simulink model "gm_PMLSM_FOC_FixedPoint_vnl"  (R2026b)
settings: Solver=FixedStepDiscrete  StopTime=0.0063  FixedStep=2e-08
undefined symbols (not defined in the file): FOC_Fixed_Config, Lookup, Ts_ACR
libraries: hdlmdlgenlib x38, simulink x16, mcbeeMathTransformLib x2
(part 2 of 6)

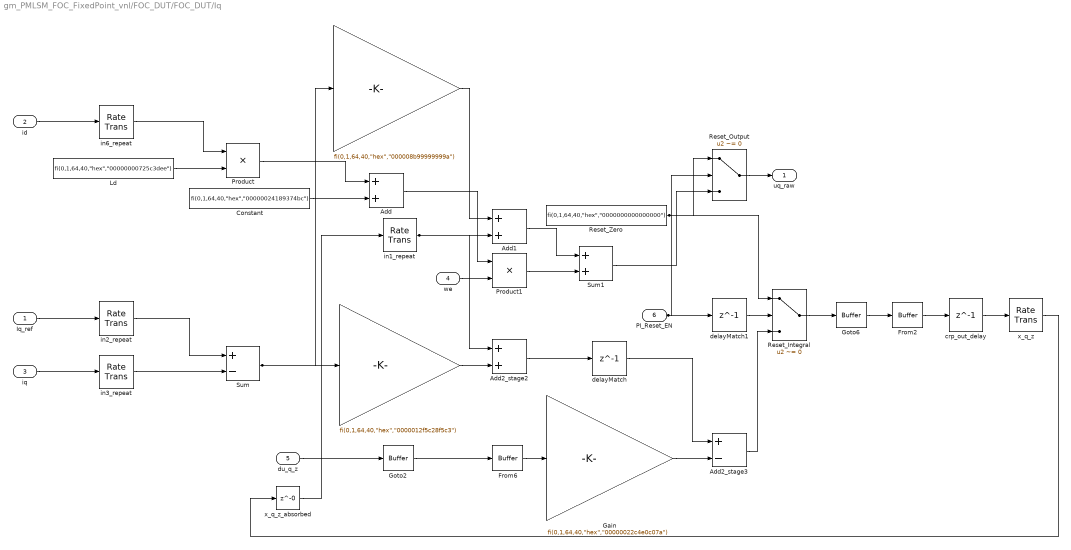
== system gm_PMLSM_FOC_FixedPoint_vnl/FOC_DUT/FOC_DUT/Iq ==
  Iq_ref : Inport  OutDataTypeStr=fixdt(1, 32, 24)  PortDimensions=1  SampleTime=0.0001
  id : Inport  Port=2  OutDataTypeStr=fixdt(1, 64, 40)  PortDimensions=1  SampleTime=0.0001
  iq : Inport  Port=3  OutDataTypeStr=fixdt(1, 64, 40)  PortDimensions=1  SampleTime=0.0001
  we : Inport  Port=4  OutDataTypeStr=fixdt(1, 40, 24)  PortDimensions=1  SampleTime=2e-08
  du_q_z : Inport  Port=5  OutDataTypeStr=fixdt(1, 64, 40)  PortDimensions=1  SampleTime=2e-08
  PI_Reset_EN : Inport  Port=6  OutDataTypeStr=boolean  PortDimensions=1  SampleTime=2e-08
  " " : Gain  Gain="fi(0,1,64,40,\"hex\",\"0000012f5c28f5c3\")"  ParamDataTypeStr=fixdt(1, 64, 40)  OutDataTypeStr=fixdt(1, 64, 40)  RndMeth=Convergent  SaturateOnIntegerOverflow=on  SampleTime=2e-08
  "  " : Gain  Gain="fi(0,1,64,40,\"hex\",\"000008b99999999a\")"  ParamDataTypeStr=fixdt(1, 64, 40)  OutDataTypeStr=fixdt(1, 64, 40)  RndMeth=Convergent  SaturateOnIntegerOverflow=on  SampleTime=2e-08
  Add : Sum  OutDataTypeStr=fixdt(1, 64, 40)  AccumDataTypeStr=fixdt(1, 64, 40)  RndMeth=Convergent  SaturateOnIntegerOverflow=on  SampleTime=2e-08
  Add1 : Sum  OutDataTypeStr=fixdt(1, 64, 40)  AccumDataTypeStr=fixdt(1, 64, 40)  RndMeth=Convergent  SaturateOnIntegerOverflow=on  SampleTime=2e-08
  Add2_stage2 : Sum  OutDataTypeStr=fixdt(1, 64, 40)  AccumDataTypeStr=fixdt(1, 64, 40)  RndMeth=Convergent  SaturateOnIntegerOverflow=on  SampleTime=2e-08
  Add2_stage3 : Sum  Inputs=+-  OutDataTypeStr=fixdt(1, 64, 40)  AccumDataTypeStr=fixdt(1, 64, 40)  RndMeth=Convergent  SaturateOnIntegerOverflow=on  SampleTime=2e-08
  Constant : Constant  Value="fi(0,1,64,40,\"hex\",\"00000024189374bc\")"  OutDataTypeStr=fixdt(1, 64, 40)  SampleTime=2e-08
  From2 : hdlmdlgenlib/Buffer
  From6 : hdlmdlgenlib/Buffer
  Gain : Gain  Gain="fi(0,1,64,40,\"hex\",\"00000022c4e0c07a\")"  ParamDataTypeStr=fixdt(1, 64, 40)  OutDataTypeStr=fixdt(1, 64, 40)  RndMeth=Convergent  SaturateOnIntegerOverflow=on  SampleTime=2e-08
  Goto2 : hdlmdlgenlib/Buffer
  Goto6 : hdlmdlgenlib/Buffer
  Ld : Constant  Value="fi(0,1,64,40,\"hex\",\"00000000725c3dee\")"  OutDataTypeStr=fixdt(1, 64, 40)  SampleTime=2e-08
  Product : Product  Inputs=**  OutDataTypeStr=fixdt(1, 64, 40)  RndMeth=Convergent  SaturateOnIntegerOverflow=on  SampleTime=2e-08
  Product1 : Product  Inputs=**  OutDataTypeStr=fixdt(1, 64, 40)  RndMeth=Convergent  SaturateOnIntegerOverflow=on  SampleTime=2e-08
  Reset_Integral : Switch  Criteria=u2 ~= 0  Threshold="fi(0,0,1,0,\"hex\",\"0\")"  OutDataTypeStr=fixdt(1, 64, 40)  RndMeth=Convergent  SampleTime=2e-08  InputSameDT=off
  Reset_Output : Switch  Criteria=u2 ~= 0  Threshold="fi(0,0,1,0,\"hex\",\"0\")"  OutDataTypeStr=fixdt(1, 64, 40)  RndMeth=Convergent  SampleTime=2e-08  InputSameDT=off
  Reset_Zero : Constant  Value="fi(0,1,64,40,\"hex\",\"0000000000000000\")"  OutDataTypeStr=fixdt(1, 64, 40)  SampleTime=2e-08
  Sum : Sum  Inputs=+-  OutDataTypeStr=fixdt(1, 64, 40)  AccumDataTypeStr=fixdt(1, 64, 40)  RndMeth=Convergent  SaturateOnIntegerOverflow=on  SampleTime=2e-08
  Sum1 : Sum  OutDataTypeStr=fixdt(1, 64, 40)  AccumDataTypeStr=fixdt(1, 64, 40)  RndMeth=Convergent  SaturateOnIntegerOverflow=on  SampleTime=2e-08
  crp_out_delay : Delay  DelayLength=1  InitialCondition=0  SampleTime=2e-08
  delayMatch : Delay  DelayLength=1  InitialCondition=0  SampleTime=2e-08
  delayMatch1 : Delay  DelayLength=1  InitialCondition=0  SampleTime=2e-08
  in1_repeat : RateTransition  Integrity=off  Deterministic=off  OutPortSampleTimeOpt=Multiple of input port sample time  OutPortSampleTimeMultiple=1/5000
  in2_repeat : RateTransition  Integrity=off  Deterministic=off  OutPortSampleTimeOpt=Multiple of input port sample time  OutPortSampleTimeMultiple=1/5000
  in3_repeat : RateTransition  Integrity=off  Deterministic=off  OutPortSampleTimeOpt=Multiple of input port sample time  OutPortSampleTimeMultiple=1/5000
  in6_repeat : RateTransition  Integrity=off  Deterministic=off  OutPortSampleTimeOpt=Multiple of input port sample time  OutPortSampleTimeMultiple=1/5000
  x_q_z : RateTransition  OutPortSampleTimeOpt=Multiple of input port sample time  OutPortSampleTimeMultiple=5000
  x_q_z_absorbed : Delay  DelayLength=0
  uq_raw : Outport  OutDataTypeStr=fixdt(1, 64, 40)  PortDimensions=1  SampleTime=2e-08
  wires:
  x_q_z/1 -> x_q_z_absorbed/1
  From2/1 -> crp_out_delay/1
  Goto6/1 -> From2/1
  Reset_Integral/1 -> Goto6/1
  Add2_stage3/1 -> Reset_Integral/3
  Gain/1 -> Add2_stage3/2
  delayMatch/1 -> Add2_stage3/1
  PI_Reset_EN/1 -> Reset_Output/2, delayMatch1/1
  Sum1/1 -> Reset_Output/3
  Reset_Zero/1 -> Reset_Output/1, Reset_Integral/1
  From6/1 -> Gain/1
  Add2_stage2/1 -> delayMatch/1
  crp_out_delay/1 -> x_q_z/1
  Product1/1 -> Sum1/2
  Add1/1 -> Sum1/1
  Goto2/1 -> From6/1
  " "/1 -> Add2_stage2/2
  we/1 -> Product1/2
  in1_repeat/1 -> Add1/2, Add2_stage2/1
  Add/1 -> Product1/1
  "  "/1 -> Add1/1
  x_q_z_absorbed/1 -> in1_repeat/1
  du_q_z/1 -> Goto2/1
  Sum/1 -> "  "/1, " "/1
  delayMatch1/1 -> Reset_Integral/2
  Constant/1 -> Add/2
  in3_repeat/1 -> Sum/2
  in2_repeat/1 -> Sum/1
  Product/1 -> Add/1
  iq/1 -> in3_repeat/1
  Iq_ref/1 -> in2_repeat/1
  Reset_Output/1 -> uq_raw/1
  in6_repeat/1 -> Product/1
  id/1 -> in6_repeat/1
  Ld/1 -> Product/2

== system gm_PMLSM_FOC_FixedPoint_vnl/FOC_DUT/FOC_DUT/Park ==
  A : Inport  OutDataTypeStr=fixdt(1,64,40,'DataTypeOverride', 'Off')  PortDimensions=1  SampleTime=0.0001
  B : Inport  Port=2  OutDataTypeStr=fixdt(1,64,40,'DataTypeOverride', 'Off')  PortDimensions=1  SampleTime=0.0001
  C : Inport  Port=3  OutDataTypeStr=fixdt(1,40,32,'DataTypeOverride', 'Off')  PortDimensions=1  SampleTime=0.0001
  Variant : Subsystem
  O1 : Outport  OutDataTypeStr=fixdt(1, 64, 40)  PortDimensions=1  SampleTime=0.0001
  O2 : Outport  Port=2  OutDataTypeStr=fixdt(1, 64, 40)  PortDimensions=1  SampleTime=0.0001
  wires:
  Variant/2(O2) -> O2/1
  C/1 -> Variant/3(C)
  B/1 -> Variant/2(B)
  A/1 -> Variant/1(A)
  Variant/1(O1) -> O1/1

== system gm_PMLSM_FOC_FixedPoint_vnl/FOC_DUT/FOC_DUT/SVPWMG ==
  Valpha : Inport  OutDataTypeStr=fixdt(1, 64, 40)  PortDimensions=1  SampleTime=2e-08
  Vbeta : Inport  Port=2  OutDataTypeStr=fixdt(1, 64, 40)  PortDimensions=1  SampleTime=2e-08
  Vdc_V : Inport  Port=3  OutDataTypeStr=fixdt(0, 32, 24)  PortDimensions=1  SampleTime=2e-08
  Duty Calculate : Subsystem
  Sector Caculate : Subsystem
  T1T2 Calculate : Subsystem
  XYZ Calculate : Subsystem
  duty_u_cmd : Outport  OutDataTypeStr=fixdt(1, 64, 40)  PortDimensions=1  SampleTime=2e-08
  duty_v_cmd : Outport  Port=2  OutDataTypeStr=fixdt(1, 64, 40)  PortDimensions=1  SampleTime=2e-08
  duty_w_cmd : Outport  Port=3  OutDataTypeStr=fixdt(1, 64, 40)  PortDimensions=1  SampleTime=2e-08
  wires:
  Duty Calculate/2(Duty_V) -> duty_v_cmd/1
  Duty Calculate/1(Duty_U) -> duty_u_cmd/1
  T1T2 Calculate/2(T2) -> Duty Calculate/3(T2)
  T1T2 Calculate/1(T1) -> Duty Calculate/2(T1)
  XYZ Calculate/1(X) -> T1T2 Calculate/2(X)
  Vdc_V/1 -> XYZ Calculate/3(Udc)
  Sector Caculate/1("N ") -> T1T2 Calculate/1(N), Duty Calculate/1(N)
  XYZ Calculate/3(Z) -> T1T2 Calculate/4(Z)
  Vbeta/1 -> XYZ Calculate/2(Ubeta), Sector Caculate/2(Ubeta)
  XYZ Calculate/2(Y) -> T1T2 Calculate/3(Y)
  Duty Calculate/3(Duty_W) -> duty_w_cmd/1
  Valpha/1 -> Sector Caculate/1(Ualpha), XYZ Calculate/1(Ualpha)

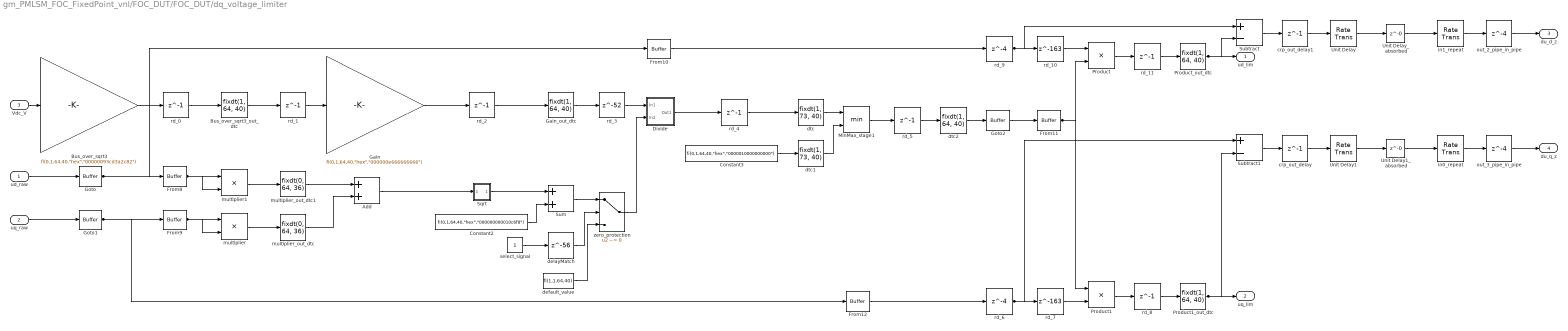
== system gm_PMLSM_FOC_FixedPoint_vnl/FOC_DUT/FOC_DUT/dq_voltage_limiter ==
  ud_raw : Inport  OutDataTypeStr=fixdt(1, 64, 40)  PortDimensions=1  SampleTime=2e-08
  uq_raw : Inport  Port=2  OutDataTypeStr=fixdt(1, 64, 40)  PortDimensions=1  SampleTime=2e-08
  Vdc_V : Inport  Port=3  OutDataTypeStr=fixdt(0, 32, 24)  PortDimensions=1  SampleTime=2e-08
  Add : Sum  OutDataTypeStr=fixdt(0, 64, 36)  AccumDataTypeStr=fixdt(0, 64, 36)  RndMeth=Convergent  SaturateOnIntegerOverflow=on  SampleTime=2e-08
  Bus_over_sqrt3 : Gain  Gain="fi(0,1,64,40,\"hex\",\"00000093cd3a2c82\")"  ParamDataTypeStr=fixdt(1, 64, 40)  OutDataTypeStr=fixdt(1, 96, 64)  SampleTime=2e-08
  Bus_over_sqrt3_out_dtc : DataTypeConversion  OutDataTypeStr=fixdt(1, 64, 40)  RndMeth=Convergent  SampleTime=2e-08
  Constant2 : Constant  Value="fi(0,1,64,40,\"hex\",\"000000000010c6f8\")"  OutDataTypeStr=fixdt(1, 64, 40)  SampleTime=2e-08
  Constant3 : Constant  Value="fi(0,1,64,40,\"hex\",\"0000010000000000\")"  OutDataTypeStr=fixdt(1, 64, 40)  SampleTime=2e-08
  Divide : Subsystem
  From{8..12} (5 alike) : hdlmdlgenlib/Buffer
  Gain : Gain  Gain="fi(0,1,64,40,\"hex\",\"000000e666666666\")"  ParamDataTypeStr=fixdt(1, 64, 40)  OutDataTypeStr=fixdt(1, 128, 80)  SampleTime=2e-08
  Gain_out_dtc : DataTypeConversion  OutDataTypeStr=fixdt(1, 64, 40)  RndMeth=Convergent  SampleTime=2e-08
  Goto : hdlmdlgenlib/Buffer
  Goto1 : hdlmdlgenlib/Buffer
  Goto2 : hdlmdlgenlib/Buffer
  MinMax_stage1 : MinMax  Inputs=2
  Product : Product  Inputs=**  OutDataTypeStr=fixdt(1, 128, 80)  SampleTime=2e-08
  Product1 : Product  Inputs=**  OutDataTypeStr=fixdt(1, 128, 80)  SampleTime=2e-08
  Product1_out_dtc : DataTypeConversion  OutDataTypeStr=fixdt(1, 64, 40)  RndMeth=Convergent  SampleTime=2e-08
  Product_out_dtc : DataTypeConversion  OutDataTypeStr=fixdt(1, 64, 40)  RndMeth=Convergent  SampleTime=2e-08
  Sqrt : Subsystem
  Subtract : Sum  Inputs=+-  OutDataTypeStr=fixdt(1, 64, 40)  AccumDataTypeStr=fixdt(1, 64, 40)  RndMeth=Convergent  SaturateOnIntegerOverflow=on  SampleTime=2e-08
  Subtract1 : Sum  Inputs=+-  OutDataTypeStr=fixdt(1, 64, 40)  AccumDataTypeStr=fixdt(1, 64, 40)  RndMeth=Convergent  SaturateOnIntegerOverflow=on  SampleTime=2e-08
  Sum : Sum  OutDataTypeStr=fixdt(1, 64, 40)  AccumDataTypeStr=fixdt(1, 64, 40)  RndMeth=Convergent  SaturateOnIntegerOverflow=on  SampleTime=2e-08
  Unit Delay : RateTransition  OutPortSampleTimeOpt=Multiple of input port sample time  OutPortSampleTimeMultiple=5000
  Unit Delay1 : RateTransition  OutPortSampleTimeOpt=Multiple of input port sample time  OutPortSampleTimeMultiple=5000
  Unit Delay1_absorbed : Delay  DelayLength=0
  Unit Delay_absorbed : Delay  DelayLength=0
  crp_out_delay : Delay  DelayLength=1  InitialCondition=0  SampleTime=2e-08
  crp_out_delay1 : Delay  DelayLength=1  InitialCondition=0  SampleTime=2e-08
  default_value : Constant  Value=fi(1,1,64,40)  OutDataTypeStr=fixdt(1, 64, 40)  SampleTime=2e-08
  delayMatch : Delay  DelayLength=56  InitialCondition=0  SampleTime=2e-08
  dtc : DataTypeConversion  OutDataTypeStr=fixdt(1, 73, 40)  RndMeth=Convergent  SampleTime=2e-08
  dtc1 : DataTypeConversion  OutDataTypeStr=fixdt(1, 73, 40)  RndMeth=Convergent  SampleTime=2e-08
  dtc2 : DataTypeConversion  OutDataTypeStr=fixdt(1, 64, 40)  RndMeth=Convergent  SampleTime=2e-08
  in0_repeat : RateTransition  Integrity=off  Deterministic=off  OutPortSampleTimeOpt=Multiple of input port sample time  OutPortSampleTimeMultiple=1/5000
  in1_repeat : RateTransition  Integrity=off  Deterministic=off  OutPortSampleTimeOpt=Multiple of input port sample time  OutPortSampleTimeMultiple=1/5000
  multiplier : Product  Inputs=**  OutDataTypeStr=fixdt(1, 128, 80)  SampleTime=2e-08
  multiplier1 : Product  Inputs=**  OutDataTypeStr=fixdt(1, 128, 80)  SampleTime=2e-08
  multiplier_out_dtc : DataTypeConversion  OutDataTypeStr=fixdt(0, 64, 36)  RndMeth=Convergent  SampleTime=2e-08
  multiplier_out_dtc1 : DataTypeConversion  OutDataTypeStr=fixdt(0, 64, 36)  RndMeth=Convergent  SampleTime=2e-08
  out_2_pipe_in_pipe : Delay  DelayLength=4  InitialCondition=0  SampleTime=2e-08
  out_3_pipe_in_pipe : Delay  DelayLength=4  InitialCondition=0  SampleTime=2e-08
  rd_{0..2,4..5,8,11} (7 alike) : Delay  DelayLength=1  InitialCondition=0  SampleTime=2e-08
  rd_10 : Delay  DelayLength=163  InitialCondition=0  SampleTime=2e-08
  rd_3 : Delay  DelayLength=52  InitialCondition=0  SampleTime=2e-08
  rd_6 : Delay  DelayLength=4  InitialCondition=0  SampleTime=2e-08
  rd_7 : Delay  DelayLength=163  InitialCondition=0  SampleTime=2e-08
  rd_9 : Delay  DelayLength=4  InitialCondition=0  SampleTime=2e-08
  select_signal : Constant  OutDataTypeStr=boolean  SampleTime=2e-08
  zero_protection : Switch  Criteria=u2 ~= 0  OutDataTypeStr=fixdt(1, 64, 40)  SampleTime=2e-08  SaturateOnIntegerOverflow=off  InputSameDT=off
  ud_lim : Outport  OutDataTypeStr=fixdt(1, 64, 40)  PortDimensions=1  SampleTime=2e-08
  uq_lim : Outport  Port=2  OutDataTypeStr=fixdt(1, 64, 40)  PortDimensions=1  SampleTime=2e-08
  du_d_z : Outport  Port=3  OutDataTypeStr=fixdt(1, 64, 40)  PortDimensions=1  SampleTime=2e-08
  du_q_z : Outport  Port=4  OutDataTypeStr=fixdt(1, 64, 40)  PortDimensions=1  SampleTime=2e-08
  wires:
  out_2_pipe_in_pipe/1 -> du_d_z/1
  in0_repeat/1 -> out_3_pipe_in_pipe/1
  in1_repeat/1 -> out_2_pipe_in_pipe/1
  crp_out_delay1/1 -> Unit Delay/1
  Subtract1/1 -> crp_out_delay/1
  Subtract/1 -> crp_out_delay1/1
  crp_out_delay/1 -> Unit Delay1/1
  Product1_out_dtc/1 -> Subtract1/2, uq_lim/1
  rd_11/1 -> Product_out_dtc/1
  rd_7/1 -> Product1/2
  Goto2/1 -> From11/1
  rd_9/1 -> rd_10/1, Subtract/1
  dtc2/1 -> Goto2/1
  rd_5/1 -> dtc2/1
  From11/1 -> Product/2, Product1/1
  From12/1 -> rd_6/1
  MinMax_stage1/1 -> rd_5/1
  out_3_pipe_in_pipe/1 -> du_q_z/1
  dtc1/1 -> MinMax_stage1/2
  Unit Delay_absorbed/1 -> in1_repeat/1
  dtc/1 -> MinMax_stage1/1
  Unit Delay1_absorbed/1 -> in0_repeat/1
  Constant3/1 -> dtc1/1
  rd_4/1 -> dtc/1
  From10/1 -> rd_9/1
  zero_protection/1 -> Divide/2(In2)
  Divide/1(Out1) -> rd_4/1
  rd_3/1 -> Divide/1(In1)
  default_value/1 -> zero_protection/3
  Product/1 -> rd_11/1
  delayMatch/1 -> zero_protection/2
  Sum/1 -> zero_protection/1
  Gain_out_dtc/1 -> rd_3/1
  select_signal/1 -> delayMatch/1
  Product1/1 -> rd_8/1
  Sqrt/1(Out1) -> Sum/1
  rd_2/1 -> Gain_out_dtc/1
  Constant2/1 -> Sum/2
  multiplier_out_dtc/1 -> Add/2
  multiplier_out_dtc1/1 -> Add/1
  rd_1/1 -> Gain/1
  multiplier/1 -> multiplier_out_dtc/1
  rd_6/1 -> rd_7/1, Subtract1/1
  multiplier1/1 -> multiplier_out_dtc1/1
  rd_10/1 -> Product/1
  Bus_over_sqrt3_out_dtc/1 -> rd_1/1
  From9/1 -> multiplier/1, multiplier/2
  rd_0/1 -> Bus_over_sqrt3_out_dtc/1
  Gain/1 -> rd_2/1
  Goto1/1 -> From9/1, From12/1
  rd_8/1 -> Product1_out_dtc/1
  From8/1 -> multiplier1/1, multiplier1/2
  Goto/1 -> From8/1, From10/1
  uq_raw/1 -> Goto1/1
  Product_out_dtc/1 -> ud_lim/1, Subtract/2
  Bus_over_sqrt3/1 -> rd_0/1
  ud_raw/1 -> Goto/1
  Add/1 -> Sqrt/1(In1)
  Unit Delay/1 -> Unit Delay_absorbed/1
  Vdc_V/1 -> Bus_over_sqrt3/1
  Unit Delay1/1 -> Unit Delay1_absorbed/1

== system gm_PMLSM_FOC_FixedPoint_vnl/FOC_DUT_vnl/SVPWMG/Duty Calculate ==
  N : Inport
  T1 : Inport  Port=2
  T2 : Inport  Port=3
  Constant : Constant  Value=FOC_Fixed_Config.Coefficients.Ts.quantized  OutDataTypeStr=FOC_Fixed_Config.Types.Work
  Fcn : Subsystem
  Fcn1 : Subsystem
  Fcn2 : Subsystem
  Gain : Gain  Gain=FOC_Fixed_Config.Coefficients.DutyGain.quantized  ParamDataTypeStr=FOC_Fixed_Config.Types.Coefficient  OutDataTypeStr=FOC_Fixed_Config.Types.Work  RndMeth=Convergent  SaturateOnIntegerOverflow=on
  Gain1 : Gain  Gain=FOC_Fixed_Config.Coefficients.DutyGain.quantized  ParamDataTypeStr=FOC_Fixed_Config.Types.Coefficient  OutDataTypeStr=FOC_Fixed_Config.Types.Work  RndMeth=Convergent  SaturateOnIntegerOverflow=on
  Gain1_UpperDuty : Bias  Bias=1
  Gain2 : Gain  Gain=FOC_Fixed_Config.Coefficients.DutyGain.quantized  ParamDataTypeStr=FOC_Fixed_Config.Types.Coefficient  OutDataTypeStr=FOC_Fixed_Config.Types.Work  RndMeth=Convergent  SaturateOnIntegerOverflow=on
  Gain2_UpperDuty : Bias  Bias=1
  Gain_UpperDuty : Bias  Bias=1
  Multiport Switch : MultiPortSwitch  Inputs=6  OutDataTypeStr=FOC_Fixed_Config.Types.Work  RndMeth=Convergent  InputSameDT=off
  Multiport Switch1 : MultiPortSwitch  Inputs=6  OutDataTypeStr=FOC_Fixed_Config.Types.Work  RndMeth=Convergent  InputSameDT=off
  Multiport Switch2 : MultiPortSwitch  Inputs=6  OutDataTypeStr=FOC_Fixed_Config.Types.Work  RndMeth=Convergent  InputSameDT=off
  Mux : Mux  Inputs=3
  Duty_U : Outport
  Duty_V : Outport  Port=2
  Duty_W : Outport  Port=3
  wires:
  Fcn2/1(Value) -> Multiport Switch2/4, Multiport Switch2/2, Multiport Switch1/7, Multiport Switch1/3, Multiport Switch/6, Multiport Switch/5
  Fcn1/1(Value) -> Multiport Switch/2, Multiport Switch/7, Multiport Switch1/4, Multiport Switch2/6, Multiport Switch2/3, Multiport Switch1/5
  Fcn/1(Value) -> Multiport Switch1/2, Multiport Switch2/7, Multiport Switch2/5, Multiport Switch1/6, Multiport Switch/4, Multiport Switch/3
  N/1 -> Multiport Switch/1, Multiport Switch1/1, Multiport Switch2/1
  Multiport Switch/1 -> Gain/1
  Multiport Switch1/1 -> Gain1/1
  Multiport Switch2/1 -> Gain2/1
  T1/1 -> Mux/1
  T2/1 -> Mux/2
  Constant/1 -> Mux/3
  Mux/1 -> Fcn2/1(Vector), Fcn1/1(Vector), Fcn/1(Vector)
  Gain/1 -> Gain_UpperDuty/1  "DutyU"
  Gain_UpperDuty/1 -> Duty_U/1
  Gain1/1 -> Gain1_UpperDuty/1  "DutyV"
  Gain1_UpperDuty/1 -> Duty_V/1
  Gain2/1 -> Gain2_UpperDuty/1  "DutyW"
  Gain2_UpperDuty/1 -> Duty_W/1

== system gm_PMLSM_FOC_FixedPoint_vnl/FOC_DUT_vnl/SVPWMG/Sector Caculate ==
  Ualpha : Inport
  Ubeta : Inport  Port=2
  B0 : Subsystem
  B1 : Subsystem
  B2 : Subsystem
  Constant : Constant  OutDataTypeStr=uint8
  Constant1 : Constant  Value=0  OutDataTypeStr=uint8
  Mux : Mux  Inputs=2
  Mux1 : Mux  Inputs=3
  N : Subsystem
  Switch : Switch  Criteria=u2 > Threshold  OutDataTypeStr=uint8  RndMeth=Convergent  InputSameDT=off
  Switch1 : Switch  OutDataTypeStr=uint8  RndMeth=Convergent  InputSameDT=off
  Switch2 : Switch  Criteria=u2 > Threshold  OutDataTypeStr=uint8  RndMeth=Convergent  InputSameDT=off
  "N " : Outport  VectorParamsAs1DForOutWhenUnconnected=off
  wires:
  N/1(Value) -> "N "/1
  Mux1/1 -> N/1(Vector)
  B2/1(Value) -> Switch2/2
  B1/1(Value) -> Switch1/2
  B0/1(Value) -> Switch/2
  Switch1/1 -> Mux1/2
  Constant1/1 -> Switch2/3, Switch1/3, Switch/3
  Constant/1 -> Switch1/1, Switch2/1, Switch/1
  Mux/1 -> B2/1(Vector), B1/1(Vector), B0/1(Vector)
  Ubeta/1 -> Mux/2
  Ualpha/1 -> Mux/1
  Switch/1 -> Mux1/1
  Switch2/1 -> Mux1/3

== system gm_PMLSM_FOC_FixedPoint_vnl/FOC_DUT_vnl/SVPWMG/T1T2 Calculate ==
  N : Inport
  X : Inport  Port=2
  Y : Inport  Port=3
  Z : Inport  Port=4
  Constant : Constant  Value=FOC_Fixed_Config.Coefficients.Ts.quantized  OutDataTypeStr=FOC_Fixed_Config.Types.Work
  Fcn : Subsystem
  Fcn1 : Subsystem
  Fcn2 : Subsystem
  Gain : Gain  Gain=-1  ParamDataTypeStr=FOC_Fixed_Config.Types.Coefficient  OutDataTypeStr=FOC_Fixed_Config.Types.Work  RndMeth=Convergent  SaturateOnIntegerOverflow=on
  Gain1 : Gain  Gain=-1  ParamDataTypeStr=FOC_Fixed_Config.Types.Coefficient  OutDataTypeStr=FOC_Fixed_Config.Types.Work  RndMeth=Convergent  SaturateOnIntegerOverflow=on
  Gain2 : Gain  Gain=-1  ParamDataTypeStr=FOC_Fixed_Config.Types.Coefficient  OutDataTypeStr=FOC_Fixed_Config.Types.Work  RndMeth=Convergent  SaturateOnIntegerOverflow=on
  Multiport Switch : MultiPortSwitch  Inputs=6  OutDataTypeStr=FOC_Fixed_Config.Types.Work  RndMeth=Convergent  InputSameDT=off
  Multiport Switch1 : MultiPortSwitch  Inputs=6  OutDataTypeStr=FOC_Fixed_Config.Types.Work  RndMeth=Convergent  InputSameDT=off
  Mux : Mux  Inputs=3
  Switch : Switch  OutDataTypeStr=FOC_Fixed_Config.Types.Work  RndMeth=Convergent  InputSameDT=off
  Switch1 : Switch  Criteria=u2 > Threshold  OutDataTypeStr=FOC_Fixed_Config.Types.Work  RndMeth=Convergent  InputSameDT=off
  T1 : Outport  VectorParamsAs1DForOutWhenUnconnected=off
  T2 : Outport  Port=2  VectorParamsAs1DForOutWhenUnconnected=off
  wires:
  Fcn/1(Value) -> Switch1/2, Switch/2
  Fcn2/1(Value) -> Switch1/3
  Fcn1/1(Value) -> Switch/3
  Gain1/1 -> Multiport Switch/7, Multiport Switch1/6
  Gain2/1 -> Multiport Switch1/7, Multiport Switch/4
  Gain/1 -> Multiport Switch/5, Multiport Switch1/3
  X/1 -> Multiport Switch1/4, Multiport Switch/6, Gain/1
  Z/1 -> Gain2/1, Multiport Switch/2, Multiport Switch1/5
  Y/1 -> Gain1/1, Multiport Switch1/2, Multiport Switch/3
  N/1 -> Multiport Switch1/1, Multiport Switch/1
  Multiport Switch1/1 -> Mux/2, Switch1/1
  Multiport Switch/1 -> Mux/1, Switch/1
  Mux/1 -> Fcn/1(Vector), Fcn2/1(Vector), Fcn1/1(Vector)
  Switch/1 -> T1/1  "T1"
  Switch1/1 -> T2/1  "T2"
  Constant/1 -> Mux/3

== system gm_PMLSM_FOC_FixedPoint_vnl/FOC_DUT_vnl/SVPWMG/XYZ Calculate ==
  Ualpha : Inport
  Ubeta : Inport  Port=2
  Udc : Inport  Port=3
  Add : Sum  OutDataTypeStr=FOC_Fixed_Config.Types.Work  AccumDataTypeStr=FOC_Fixed_Config.Types.Work  RndMeth=Convergent  SaturateOnIntegerOverflow=on
  Add1 : Sum  Inputs=+-  OutDataTypeStr=FOC_Fixed_Config.Types.Work  AccumDataTypeStr=FOC_Fixed_Config.Types.Work  RndMeth=Convergent  SaturateOnIntegerOverflow=on
  Constant1 : Constant  Value=FOC_Fixed_Config.Coefficients.Ts.quantized  OutDataTypeStr=FOC_Fixed_Config.Types.Work
  Gain : Gain  Gain=3/2  ParamDataTypeStr=FOC_Fixed_Config.Types.Coefficient  OutDataTypeStr=FOC_Fixed_Config.Types.Work  RndMeth=Convergent  SaturateOnIntegerOverflow=on
  Gain1 : Gain  Gain=FOC_Fixed_Config.Coefficients.C17321.quantized  ParamDataTypeStr=FOC_Fixed_Config.Types.Coefficient  OutDataTypeStr=FOC_Fixed_Config.Types.Work  RndMeth=Convergent  SaturateOnIntegerOverflow=on
  Gain2 : Gain  Gain=FOC_Fixed_Config.Coefficients.C0866.quantized  ParamDataTypeStr=FOC_Fixed_Config.Types.Coefficient  OutDataTypeStr=FOC_Fixed_Config.Types.Work  RndMeth=Convergent  SaturateOnIntegerOverflow=on
  Math Function : Math  Operator=reciprocal  OutDataTypeStr=FOC_Fixed_Config.Types.Work  RndMeth=Convergent
  Product{,1..3} (4 alike) : Product  OutDataTypeStr=FOC_Fixed_Config.Types.Work  RndMeth=Convergent  SaturateOnIntegerOverflow=on
  X : Outport
  Y : Outport  Port=2
  Z : Outport  Port=3
  wires:
  Constant1/1 -> Product/1
  Product3/1 -> Y/1  "Y"
  Product2/1 -> Z/1  "Z"
  Add1/1 -> Product2/1
  Add/1 -> Product3/1
  Product1/1 -> X/1  "X"
  Gain/1 -> Add/2, Add1/2
  Gain2/1 -> Add1/1, Add/1
  Product/1 -> Product1/2, Product3/2, Product2/2
  Gain1/1 -> Product1/1
  Ubeta/1 -> Gain1/1, Gain2/1
  Math Function/1 -> Product/2
  Udc/1 -> Math Function/1
  Ualpha/1 -> Gain/1

== system gm_PMLSM_FOC_FixedPoint_vnl/FOC_DUT/FOC_DUT/InversePark/Variant ==
  A : Inport  OutDataTypeStr=fixdt(1, 64, 40)  PortDimensions=1  SampleTime=2e-08
  B : Inport  Port=2  OutDataTypeStr=fixdt(1, 64, 40)  PortDimensions=1  SampleTime=2e-08
  C : Inport  Port=3  OutDataTypeStr=fixdt(1, 40, 32)  PortDimensions=1  SampleTime=0.0001
  mcb : Subsystem
  O1 : Outport  OutDataTypeStr=fixdt(1, 64, 40)  PortDimensions=1  SampleTime=2e-08
  O2 : Outport  Port=2  OutDataTypeStr=fixdt(1, 64, 40)  PortDimensions=1  SampleTime=2e-08
  wires:
  mcb/2(O2) -> O2/1
  mcb/1(O1) -> O1/1
  C/1 -> mcb/3(C)
  B/1 -> mcb/2(B)
  A/1 -> mcb/1(A)

== system gm_PMLSM_FOC_FixedPoint_vnl/FOC_DUT/FOC_DUT/Park/Variant ==
  A : Inport  OutDataTypeStr=fixdt(1, 64, 40)  PortDimensions=1  SampleTime=0.0001
  B : Inport  Port=2  OutDataTypeStr=fixdt(1, 64, 40)  PortDimensions=1  SampleTime=0.0001
  C : Inport  Port=3  OutDataTypeStr=fixdt(1, 40, 32)  PortDimensions=1  SampleTime=0.0001
  mcb : Subsystem
  O1 : Outport  OutDataTypeStr=fixdt(1, 64, 40)  PortDimensions=1  SampleTime=0.0001
  O2 : Outport  Port=2  OutDataTypeStr=fixdt(1, 64, 40)  PortDimensions=1  SampleTime=0.0001
  wires:
  mcb/2(O2) -> O2/1
  mcb/1(O1) -> O1/1
  C/1 -> mcb/3(C)
  B/1 -> mcb/2(B)
  A/1 -> mcb/1(A)

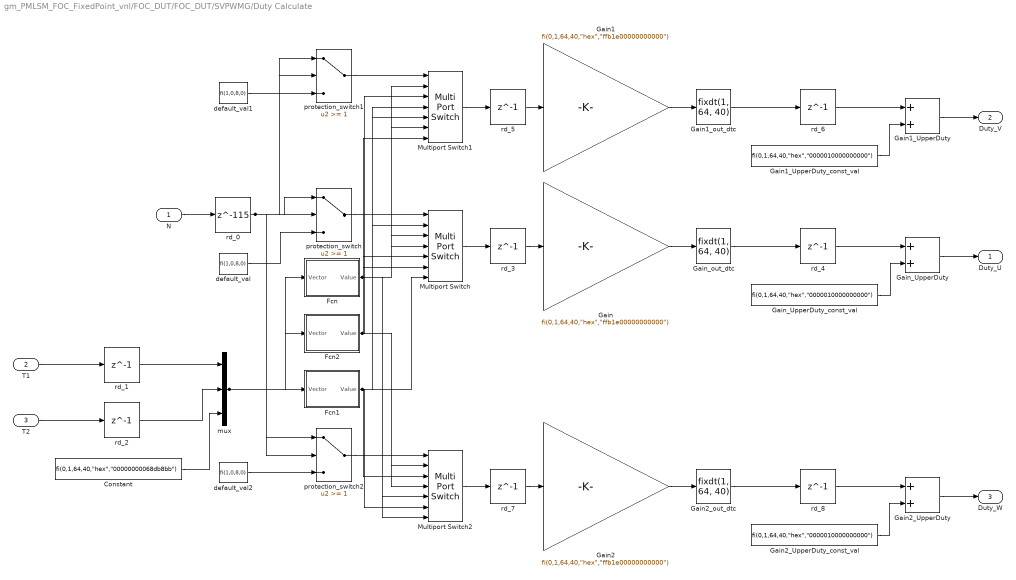
== system gm_PMLSM_FOC_FixedPoint_vnl/FOC_DUT/FOC_DUT/SVPWMG/Duty Calculate ==
  N : Inport  OutDataTypeStr=uint8  PortDimensions=1  SampleTime=2e-08
  T1 : Inport  Port=2  OutDataTypeStr=fixdt(1, 64, 40)  PortDimensions=1  SampleTime=2e-08
  T2 : Inport  Port=3  OutDataTypeStr=fixdt(1, 64, 40)  PortDimensions=1  SampleTime=2e-08
  Constant : Constant  Value="fi(0,1,64,40,\"hex\",\"00000000068db8bb\")"  OutDataTypeStr=fixdt(1, 64, 40)  SampleTime=2e-08
  Fcn : Subsystem
  Fcn1 : Subsystem
  Fcn2 : Subsystem
  Gain : Gain  Gain="fi(0,1,64,40,\"hex\",\"ffb1e00000000000\")"  ParamDataTypeStr=fixdt(1, 64, 40)  OutDataTypeStr=fixdt(1, 128, 80)  SampleTime=2e-08
  Gain1 : Gain  Gain="fi(0,1,64,40,\"hex\",\"ffb1e00000000000\")"  ParamDataTypeStr=fixdt(1, 64, 40)  OutDataTypeStr=fixdt(1, 128, 80)  SampleTime=2e-08
  Gain1_UpperDuty : Sum  OutDataTypeStr=fixdt(1, 64, 40)  AccumDataTypeStr=fixdt(1, 64, 40)  RndMeth=Nearest  SaturateOnIntegerOverflow=on  SampleTime=2e-08
  Gain1_UpperDuty_const_val : Constant  Value="fi(0,1,64,40,\"hex\",\"0000010000000000\")"  VectorParams1D=off  OutDataTypeStr=fixdt(1, 64, 40)  SampleTime=2e-08
  Gain1_out_dtc : DataTypeConversion  OutDataTypeStr=fixdt(1, 64, 40)  RndMeth=Convergent  SampleTime=2e-08
  Gain2 : Gain  Gain="fi(0,1,64,40,\"hex\",\"ffb1e00000000000\")"  ParamDataTypeStr=fixdt(1, 64, 40)  OutDataTypeStr=fixdt(1, 128, 80)  SampleTime=2e-08
  Gain2_UpperDuty : Sum  OutDataTypeStr=fixdt(1, 64, 40)  AccumDataTypeStr=fixdt(1, 64, 40)  RndMeth=Nearest  SaturateOnIntegerOverflow=on  SampleTime=2e-08
  Gain2_UpperDuty_const_val : Constant  Value="fi(0,1,64,40,\"hex\",\"0000010000000000\")"  VectorParams1D=off  OutDataTypeStr=fixdt(1, 64, 40)  SampleTime=2e-08
  Gain2_out_dtc : DataTypeConversion  OutDataTypeStr=fixdt(1, 64, 40)  RndMeth=Convergent  SampleTime=2e-08
  Gain_UpperDuty : Sum  OutDataTypeStr=fixdt(1, 64, 40)  AccumDataTypeStr=fixdt(1, 64, 40)  RndMeth=Nearest  SaturateOnIntegerOverflow=on  SampleTime=2e-08
  Gain_UpperDuty_const_val : Constant  Value="fi(0,1,64,40,\"hex\",\"0000010000000000\")"  VectorParams1D=off  OutDataTypeStr=fixdt(1, 64, 40)  SampleTime=2e-08
  Gain_out_dtc : DataTypeConversion  OutDataTypeStr=fixdt(1, 64, 40)  RndMeth=Convergent  SampleTime=2e-08
  Multiport Switch : MultiPortSwitch  Inputs=6  DiagnosticForDefault=None  OutDataTypeStr=fixdt(1, 64, 40)  RndMeth=Convergent  SampleTime=2e-08  InputSameDT=off
  Multiport Switch1 : MultiPortSwitch  Inputs=6  DiagnosticForDefault=None  OutDataTypeStr=fixdt(1, 64, 40)  RndMeth=Convergent  SampleTime=2e-08  InputSameDT=off
  Multiport Switch2 : MultiPortSwitch  Inputs=6  DiagnosticForDefault=None  OutDataTypeStr=fixdt(1, 64, 40)  RndMeth=Convergent  SampleTime=2e-08  InputSameDT=off
  default_val : Constant  Value=fi(1,0,8,0)  OutDataTypeStr=uint8  SampleTime=2e-08
  default_val1 : Constant  Value=fi(1,0,8,0)  OutDataTypeStr=uint8  SampleTime=2e-08
  default_val2 : Constant  Value=fi(1,0,8,0)  OutDataTypeStr=uint8  SampleTime=2e-08
  mux : Mux  Inputs=3
  protection_switch : Switch  Threshold=1  OutDataTypeStr=uint8  SampleTime=2e-08  SaturateOnIntegerOverflow=off  InputSameDT=off
  protection_switch1 : Switch  Threshold=1  OutDataTypeStr=uint8  SampleTime=2e-08  SaturateOnIntegerOverflow=off  InputSameDT=off
  protection_switch2 : Switch  Threshold=1  OutDataTypeStr=uint8  SampleTime=2e-08  SaturateOnIntegerOverflow=off  InputSameDT=off
  rd_0 : Delay  DelayLength=115  InitialCondition=0  SampleTime=2e-08
  rd_{1..8} (8 alike) : Delay  DelayLength=1  InitialCondition=0  SampleTime=2e-08
  Duty_U : Outport  OutDataTypeStr=fixdt(1, 64, 40)  PortDimensions=1  SampleTime=2e-08
  Duty_V : Outport  Port=2  OutDataTypeStr=fixdt(1, 64, 40)  PortDimensions=1  SampleTime=2e-08
  Duty_W : Outport  Port=3  OutDataTypeStr=fixdt(1, 64, 40)  PortDimensions=1  SampleTime=2e-08
  wires:
  Gain2_UpperDuty_const_val/1 -> Gain2_UpperDuty/2
  Gain_UpperDuty_const_val/1 -> Gain_UpperDuty/2
  rd_4/1 -> Gain_UpperDuty/1
  Gain_UpperDuty/1 -> Duty_U/1
  rd_6/1 -> Gain1_UpperDuty/1
  Gain2_UpperDuty/1 -> Duty_W/1
  Gain_out_dtc/1 -> rd_4/1
  Gain2/1 -> Gain2_out_dtc/1
  Gain2_out_dtc/1 -> rd_8/1
  Gain1/1 -> Gain1_out_dtc/1
  rd_3/1 -> Gain/1
  rd_5/1 -> Gain1/1
  Gain1_UpperDuty/1 -> Duty_V/1
  Multiport Switch2/1 -> rd_7/1
  Gain/1 -> Gain_out_dtc/1
  protection_switch2/1 -> Multiport Switch2/1
  Fcn1/1(Value) -> Multiport Switch2/6, Multiport Switch1/5, Multiport Switch/2, Multiport Switch/7, Multiport Switch1/4, Multiport Switch2/3
  Fcn2/1(Value) -> Multiport Switch2/4, Multiport Switch1/3, Multiport Switch/5, Multiport Switch/6, Multiport Switch1/7, Multiport Switch2/2
  Fcn/1(Value) -> Multiport Switch1/2, Multiport Switch/3, Multiport Switch/4, Multiport Switch1/6, Multiport Switch2/5, Multiport Switch2/7
  protection_switch/1 -> Multiport Switch/1
  default_val2/1 -> protection_switch2/3
  Multiport Switch1/1 -> rd_5/1
  mux/1 -> Fcn2/1(Vector), Fcn1/1(Vector), Fcn/1(Vector)
  Gain1_out_dtc/1 -> rd_6/1
  default_val/1 -> protection_switch/3
  rd_0/1 -> protection_switch/2, protection_switch2/2, protection_switch/1, protection_switch1/2, protection_switch2/1, protection_switch1/1
  default_val1/1 -> protection_switch1/3
  rd_2/1 -> mux/2
  Multiport Switch/1 -> rd_3/1
  rd_1/1 -> mux/1
  N/1 -> rd_0/1
  rd_7/1 -> Gain2/1
  Constant/1 -> mux/3
  protection_switch1/1 -> Multiport Switch1/1
  T2/1 -> rd_2/1
  rd_8/1 -> Gain2_UpperDuty/1
  T1/1 -> rd_1/1
  Gain1_UpperDuty_const_val/1 -> Gain1_UpperDuty/2

== system gm_PMLSM_FOC_FixedPoint_vnl/FOC_DUT/FOC_DUT/SVPWMG/Sector Caculate ==
  Ualpha : Inport  OutDataTypeStr=fixdt(1, 64, 40)  PortDimensions=1  SampleTime=2e-08
  Ubeta : Inport  Port=2  OutDataTypeStr=fixdt(1, 64, 40)  PortDimensions=1  SampleTime=2e-08
  B0 : Subsystem
  B1 : Subsystem
  B2 : Subsystem
  Constant : Constant  OutDataTypeStr=uint8  SampleTime=2e-08
  Constant1 : Constant  Value=0  OutDataTypeStr=uint8  SampleTime=2e-08
  N : Subsystem
  Switch : Switch  Criteria=u2 > Threshold  Threshold="fi(0,1,64,40,\"hex\",\"0000000000000000\")"  OutDataTypeStr=uint8  RndMeth=Convergent  SampleTime=2e-08  InputSameDT=off
  Switch1 : Switch  Threshold="fi(0,1,64,40,\"hex\",\"0000000000000000\")"  OutDataTypeStr=uint8  RndMeth=Convergent  SampleTime=2e-08  InputSameDT=off
  Switch2 : Switch  Criteria=u2 > Threshold  Threshold="fi(0,1,64,40,\"hex\",\"0000000000000000\")"  OutDataTypeStr=uint8  RndMeth=Convergent  SampleTime=2e-08  InputSameDT=off
  mux : Mux  Inputs=2
  mux1 : Mux  Inputs=3
  rd_0 : Delay  DelayLength=1  InitialCondition=0  SampleTime=2e-08
  "N " : Outport  OutDataTypeStr=uint8  PortDimensions=1  SampleTime=2e-08  VectorParamsAs1DForOutWhenUnconnected=off
  wires:
  mux1/1 -> N/1(Vector)
  rd_0/1 -> mux1/1
  Switch2/1 -> mux1/3
  Switch/1 -> rd_0/1
  Switch1/1 -> mux1/2
  B1/1(Value) -> Switch1/2
  Constant1/1 -> Switch/3, Switch1/3, Switch2/3
  B0/1(Value) -> Switch/2
  mux/1 -> B2/1(Vector), B1/1(Vector), B0/1(Vector)
  N/1(Value) -> "N "/1
  B2/1(Value) -> Switch2/2
  Constant/1 -> Switch/1, Switch1/1, Switch2/1
  Ubeta/1 -> mux/2
  Ualpha/1 -> mux/1

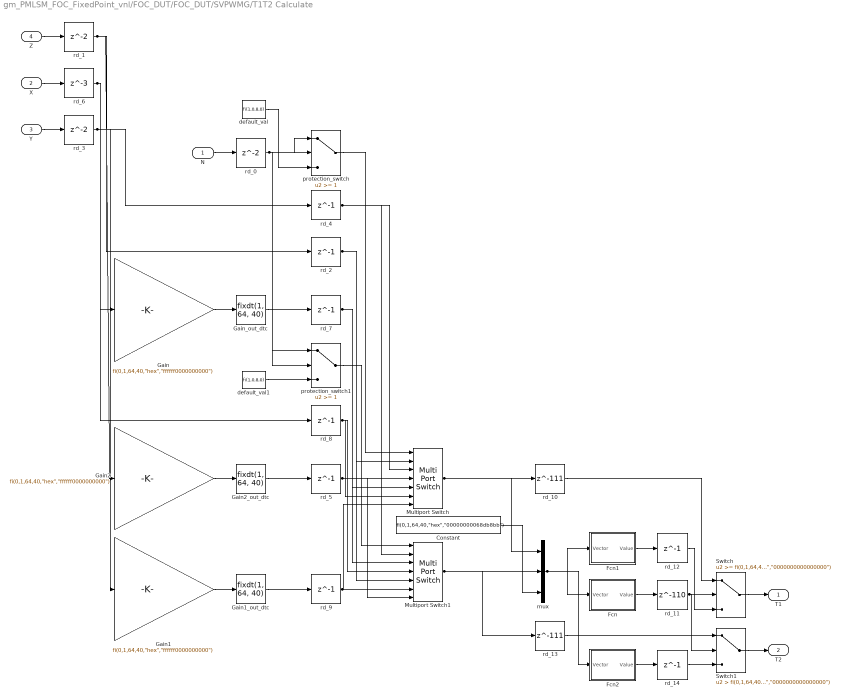
== system gm_PMLSM_FOC_FixedPoint_vnl/FOC_DUT/FOC_DUT/SVPWMG/T1T2 Calculate ==
  N : Inport  OutDataTypeStr=uint8  PortDimensions=1  SampleTime=2e-08
  X : Inport  Port=2  OutDataTypeStr=fixdt(1, 64, 40)  PortDimensions=1  SampleTime=2e-08
  Y : Inport  Port=3  OutDataTypeStr=fixdt(1, 64, 40)  PortDimensions=1  SampleTime=2e-08
  Z : Inport  Port=4  OutDataTypeStr=fixdt(1, 64, 40)  PortDimensions=1  SampleTime=2e-08
  Constant : Constant  Value="fi(0,1,64,40,\"hex\",\"00000000068db8bb\")"  OutDataTypeStr=fixdt(1, 64, 40)  SampleTime=2e-08
  Fcn : Subsystem
  Fcn1 : Subsystem
  Fcn2 : Subsystem
  Gain : Gain  Gain="fi(0,1,64,40,\"hex\",\"ffffff0000000000\")"  ParamDataTypeStr=fixdt(1, 64, 40)  OutDataTypeStr=fixdt(1, 128, 80)  SampleTime=2e-08
  Gain1 : Gain  Gain="fi(0,1,64,40,\"hex\",\"ffffff0000000000\")"  ParamDataTypeStr=fixdt(1, 64, 40)  OutDataTypeStr=fixdt(1, 128, 80)  SampleTime=2e-08
  Gain1_out_dtc : DataTypeConversion  OutDataTypeStr=fixdt(1, 64, 40)  RndMeth=Convergent  SampleTime=2e-08
  Gain2 : Gain  Gain="fi(0,1,64,40,\"hex\",\"ffffff0000000000\")"  ParamDataTypeStr=fixdt(1, 64, 40)  OutDataTypeStr=fixdt(1, 128, 80)  SampleTime=2e-08
  Gain2_out_dtc : DataTypeConversion  OutDataTypeStr=fixdt(1, 64, 40)  RndMeth=Convergent  SampleTime=2e-08
  Gain_out_dtc : DataTypeConversion  OutDataTypeStr=fixdt(1, 64, 40)  RndMeth=Convergent  SampleTime=2e-08
  Multiport Switch : MultiPortSwitch  Inputs=6  DiagnosticForDefault=None  OutDataTypeStr=fixdt(1, 64, 40)  RndMeth=Convergent  SampleTime=2e-08  InputSameDT=off
  Multiport Switch1 : MultiPortSwitch  Inputs=6  DiagnosticForDefault=None  OutDataTypeStr=fixdt(1, 64, 40)  RndMeth=Convergent  SampleTime=2e-08  InputSameDT=off
  Switch : Switch  Threshold="fi(0,1,64,40,\"hex\",\"0000000000000000\")"  OutDataTypeStr=fixdt(1, 64, 40)  RndMeth=Convergent  SampleTime=2e-08  InputSameDT=off
  Switch1 : Switch  Criteria=u2 > Threshold  Threshold="fi(0,1,64,40,\"hex\",\"0000000000000000\")"  OutDataTypeStr=fixdt(1, 64, 40)  RndMeth=Convergent  SampleTime=2e-08  InputSameDT=off
  default_val : Constant  Value=fi(1,0,8,0)  OutDataTypeStr=uint8  SampleTime=2e-08
  default_val1 : Constant  Value=fi(1,0,8,0)  OutDataTypeStr=uint8  SampleTime=2e-08
  mux : Mux  Inputs=3
  protection_switch : Switch  Threshold=1  OutDataTypeStr=uint8  SampleTime=2e-08  SaturateOnIntegerOverflow=off  InputSameDT=off
  protection_switch1 : Switch  Threshold=1  OutDataTypeStr=uint8  SampleTime=2e-08  SaturateOnIntegerOverflow=off  InputSameDT=off
  rd_0 : Delay  InitialCondition=0  SampleTime=2e-08
  rd_1 : Delay  InitialCondition=0  SampleTime=2e-08
  rd_10 : Delay  DelayLength=111  InitialCondition=0  SampleTime=2e-08
  rd_11 : Delay  DelayLength=110  InitialCondition=0  SampleTime=2e-08
  rd_{2,4..5,7..9,12,14} (8 alike) : Delay  DelayLength=1  InitialCondition=0  SampleTime=2e-08
  rd_13 : Delay  DelayLength=111  InitialCondition=0  SampleTime=2e-08
  rd_3 : Delay  InitialCondition=0  SampleTime=2e-08
  rd_6 : Delay  DelayLength=3  InitialCondition=0  SampleTime=2e-08
  T1 : Outport  OutDataTypeStr=fixdt(1, 64, 40)  PortDimensions=1  SampleTime=2e-08  VectorParamsAs1DForOutWhenUnconnected=off
  T2 : Outport  Port=2  OutDataTypeStr=fixdt(1, 64, 40)  PortDimensions=1  SampleTime=2e-08  VectorParamsAs1DForOutWhenUnconnected=off
  wires:
  Switch/1 -> T1/1
  rd_14/1 -> Switch1/3
  rd_11/1 -> Switch1/2, Switch/2
  Fcn1/1(Value) -> rd_12/1
  mux/1 -> Fcn/1(Vector), Fcn2/1(Vector), Fcn1/1(Vector)
  Multiport Switch1/1 -> rd_13/1, mux/2
  Constant/1 -> mux/3
  Multiport Switch/1 -> rd_10/1, mux/1
  rd_9/1 -> Multiport Switch/7, Multiport Switch1/6
  rd_5/1 -> Multiport Switch1/7, Multiport Switch/4
  Fcn/1(Value) -> rd_11/1
  rd_8/1 -> Multiport Switch/6, Multiport Switch1/4
  protection_switch1/1 -> Multiport Switch1/1
  rd_7/1 -> Multiport Switch1/3, Multiport Switch/5
  rd_2/1 -> Multiport Switch/2, Multiport Switch1/5
  rd_4/1 -> Multiport Switch/3, Multiport Switch1/2
  protection_switch/1 -> Multiport Switch/1
  Gain1_out_dtc/1 -> rd_9/1
  Gain2_out_dtc/1 -> rd_5/1
  Fcn2/1(Value) -> rd_14/1
  default_val1/1 -> protection_switch1/3
  Gain_out_dtc/1 -> rd_7/1
  rd_0/1 -> protection_switch/2, protection_switch1/1, protection_switch/1, protection_switch1/2
  default_val/1 -> protection_switch/3
  Gain1/1 -> Gain1_out_dtc/1
  rd_10/1 -> Switch/1
  N/1 -> rd_0/1
  Gain2/1 -> Gain2_out_dtc/1
  rd_3/1 -> Gain1/1, rd_4/1
  rd_1/1 -> rd_2/1, Gain2/1
  Gain/1 -> Gain_out_dtc/1
  rd_12/1 -> Switch/3
  Y/1 -> rd_3/1
  Switch1/1 -> T2/1
  rd_6/1 -> Gain/1, rd_8/1
  X/1 -> rd_6/1
  Z/1 -> rd_1/1
  rd_13/1 -> Switch1/1

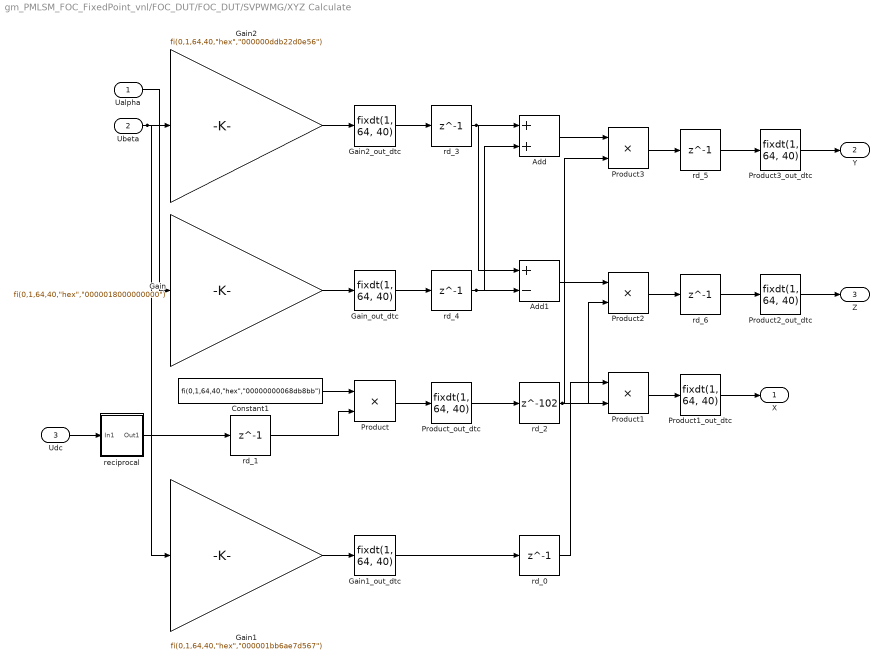
== system gm_PMLSM_FOC_FixedPoint_vnl/FOC_DUT/FOC_DUT/SVPWMG/XYZ Calculate ==
  Ualpha : Inport  OutDataTypeStr=fixdt(1, 64, 40)  PortDimensions=1  SampleTime=2e-08
  Ubeta : Inport  Port=2  OutDataTypeStr=fixdt(1, 64, 40)  PortDimensions=1  SampleTime=2e-08
  Udc : Inport  Port=3  OutDataTypeStr=fixdt(0, 32, 24)  PortDimensions=1  SampleTime=2e-08
  Add : Sum  OutDataTypeStr=fixdt(1, 64, 40)  AccumDataTypeStr=fixdt(1, 64, 40)  RndMeth=Convergent  SaturateOnIntegerOverflow=on  SampleTime=2e-08
  Add1 : Sum  Inputs=+-  OutDataTypeStr=fixdt(1, 64, 40)  AccumDataTypeStr=fixdt(1, 64, 40)  RndMeth=Convergent  SaturateOnIntegerOverflow=on  SampleTime=2e-08
  Constant1 : Constant  Value="fi(0,1,64,40,\"hex\",\"00000000068db8bb\")"  OutDataTypeStr=fixdt(1, 64, 40)  SampleTime=2e-08
  Gain : Gain  Gain="fi(0,1,64,40,\"hex\",\"0000018000000000\")"  ParamDataTypeStr=fixdt(1, 64, 40)  OutDataTypeStr=fixdt(1, 128, 80)  SampleTime=2e-08
  Gain1 : Gain  Gain="fi(0,1,64,40,\"hex\",\"000001bb6ae7d567\")"  ParamDataTypeStr=fixdt(1, 64, 40)  OutDataTypeStr=fixdt(1, 128, 80)  SampleTime=2e-08
  Gain1_out_dtc : DataTypeConversion  OutDataTypeStr=fixdt(1, 64, 40)  RndMeth=Convergent  SampleTime=2e-08
  Gain2 : Gain  Gain="fi(0,1,64,40,\"hex\",\"000000ddb22d0e56\")"  ParamDataTypeStr=fixdt(1, 64, 40)  OutDataTypeStr=fixdt(1, 128, 80)  SampleTime=2e-08
  Gain2_out_dtc : DataTypeConversion  OutDataTypeStr=fixdt(1, 64, 40)  RndMeth=Convergent  SampleTime=2e-08
  Gain_out_dtc : DataTypeConversion  OutDataTypeStr=fixdt(1, 64, 40)  RndMeth=Convergent  SampleTime=2e-08
  Product{,1..3} (4 alike) : Product  Inputs=**  OutDataTypeStr=fixdt(1, 128, 80)  SampleTime=2e-08
  Product1_out_dtc : DataTypeConversion  OutDataTypeStr=fixdt(1, 64, 40)  RndMeth=Convergent  SampleTime=2e-08
  Product2_out_dtc : DataTypeConversion  OutDataTypeStr=fixdt(1, 64, 40)  RndMeth=Convergent  SampleTime=2e-08
  Product3_out_dtc : DataTypeConversion  OutDataTypeStr=fixdt(1, 64, 40)  RndMeth=Convergent  SampleTime=2e-08
  Product_out_dtc : DataTypeConversion  OutDataTypeStr=fixdt(1, 64, 40)  RndMeth=Convergent  SampleTime=2e-08
  rd_{0..1,3..6} (6 alike) : Delay  DelayLength=1  InitialCondition=0  SampleTime=2e-08
  rd_2 : Delay  DelayLength=102  InitialCondition=0  SampleTime=2e-08
  reciprocal : Subsystem
  X : Outport  OutDataTypeStr=fixdt(1, 64, 40)  PortDimensions=1  SampleTime=2e-08
  Y : Outport  Port=2  OutDataTypeStr=fixdt(1, 64, 40)  PortDimensions=1  SampleTime=2e-08
  Z : Outport  Port=3  OutDataTypeStr=fixdt(1, 64, 40)  PortDimensions=1  SampleTime=2e-08
  wires:
  Product2_out_dtc/1 -> Z/1
  Product3_out_dtc/1 -> Y/1
  rd_6/1 -> Product2_out_dtc/1
  Product1_out_dtc/1 -> X/1
  rd_5/1 -> Product3_out_dtc/1
  Product2/1 -> rd_6/1
  Product3/1 -> rd_5/1
  rd_0/1 -> Product1/1
  rd_2/1 -> Product2/2, Product3/2, Product1/2
  Add1/1 -> Product2/1
  Product1/1 -> Product1_out_dtc/1
  Add/1 -> Product3/1
  Product_out_dtc/1 -> rd_2/1
  rd_4/1 -> Add/2, Add1/2
  Product/1 -> Product_out_dtc/1
  Gain_out_dtc/1 -> rd_4/1
  Gain2_out_dtc/1 -> rd_3/1
  Gain1/1 -> Gain1_out_dtc/1
  Constant1/1 -> Product/1
  Gain/1 -> Gain_out_dtc/1
  rd_1/1 -> Product/2
  reciprocal/1(Out1) -> rd_1/1
  Gain1_out_dtc/1 -> rd_0/1
  Gain2/1 -> Gain2_out_dtc/1
  Ubeta/1 -> Gain1/1, Gain2/1
  Ualpha/1 -> Gain/1
  Udc/1 -> reciprocal/1(In1)
  rd_3/1 -> Add/1, Add1/1

== system gm_PMLSM_FOC_FixedPoint_vnl/FOC_DUT/FOC_DUT/dq_voltage_limiter/Divide ==
  In1 : Inport
  In2 : Inport  Port=2
  Divide : Product  Inputs=*/  OutDataTypeStr=FOC_Fixed_Config.Types.DivideWide  RndMeth=Convergent  SaturateOnIntegerOverflow=on
  Divide_pd1 : Delay  DelayLength=109
  Out1 : Outport
  wires:
  Divide/1 -> Divide_pd1/1
  In2/1 -> Divide/2
  In1/1 -> Divide/1
  Divide_pd1/1 -> Out1/1

== system gm_PMLSM_FOC_FixedPoint_vnl/FOC_DUT/FOC_DUT/dq_voltage_limiter/Sqrt ==
  In1 : Inport
  Delay2 : Delay  DelayLength=56
  Sqrt : Sqrt  OutDataTypeStr=FOC_Fixed_Config.Types.Work
  Out1 : Outport
  wires:
  Delay2/1 -> Out1/1
  Sqrt/1 -> Delay2/1
  In1/1 -> Sqrt/1

== system gm_PMLSM_FOC_FixedPoint_vnl/FOC_DUT_vnl/SVPWMG/Duty Calculate/Fcn ==
  Vector : Inport
  Combination : Sum  Inputs=+--  OutDataTypeStr=FOC_Fixed_Config.Types.Work  AccumDataTypeStr=FOC_Fixed_Config.Types.Work  RndMeth=Convergent  SaturateOnIntegerOverflow=on
  Elements : Demux  Outputs=3
  Quarter : Gain  Gain=.25  ParamDataTypeStr=FOC_Fixed_Config.Types.Coefficient  OutDataTypeStr=FOC_Fixed_Config.Types.Work  RndMeth=Convergent  SaturateOnIntegerOverflow=on
  Value : Outport
  wires:
  Quarter/1 -> Value/1
  Combination/1 -> Quarter/1
  Elements/3 -> Combination/1
  Elements/1 -> Combination/2
  Elements/2 -> Combination/3
  Vector/1 -> Elements/1

== system gm_PMLSM_FOC_FixedPoint_vnl/FOC_DUT_vnl/SVPWMG/Duty Calculate/Fcn1 ==
  Vector : Inport
  Combination : Sum  Inputs=++-  OutDataTypeStr=FOC_Fixed_Config.Types.Work  AccumDataTypeStr=FOC_Fixed_Config.Types.Work  RndMeth=Convergent  SaturateOnIntegerOverflow=on
  Elements : Demux  Outputs=3
  Quarter : Gain  Gain=.25  ParamDataTypeStr=FOC_Fixed_Config.Types.Coefficient  OutDataTypeStr=FOC_Fixed_Config.Types.Work  RndMeth=Convergent  SaturateOnIntegerOverflow=on
  Value : Outport
  wires:
  Quarter/1 -> Value/1
  Combination/1 -> Quarter/1
  Elements/2 -> Combination/3
  Elements/3 -> Combination/1
  Elements/1 -> Combination/2
  Vector/1 -> Elements/1

== system gm_PMLSM_FOC_FixedPoint_vnl/FOC_DUT_vnl/SVPWMG/Duty Calculate/Fcn2 ==
  Vector : Inport
  Combination : Sum  Inputs=+++  OutDataTypeStr=FOC_Fixed_Config.Types.Work  AccumDataTypeStr=FOC_Fixed_Config.Types.Work  RndMeth=Convergent  SaturateOnIntegerOverflow=on
  Elements : Demux  Outputs=3
  Quarter : Gain  Gain=.25  ParamDataTypeStr=FOC_Fixed_Config.Types.Coefficient  OutDataTypeStr=FOC_Fixed_Config.Types.Work  RndMeth=Convergent  SaturateOnIntegerOverflow=on
  Value : Outport
  wires:
  Quarter/1 -> Value/1
  Combination/1 -> Quarter/1
  Elements/2 -> Combination/2
  Elements/3 -> Combination/1
  Elements/1 -> Combination/3
  Vector/1 -> Elements/1

== system gm_PMLSM_FOC_FixedPoint_vnl/FOC_DUT_vnl/SVPWMG/Sector Caculate/B0 ==
  Vector : Inport
  Elements : Demux  Outputs=2
  Unused_Vector_Element : Terminator
  Value : Outport
  wires:
  Elements/1 -> Unused_Vector_Element/1
  Elements/2 -> Value/1
  Vector/1 -> Elements/1

== system gm_PMLSM_FOC_FixedPoint_vnl/FOC_DUT_vnl/SVPWMG/Sector Caculate/B1 ==
  Vector : Inport
  Alpha0866 : Gain  Gain=FOC_Fixed_Config.Coefficients.C0866.quantized  ParamDataTypeStr=FOC_Fixed_Config.Types.Coefficient  OutDataTypeStr=FOC_Fixed_Config.Types.Work  RndMeth=Convergent  SaturateOnIntegerOverflow=on
  Beta05 : Gain  Gain=0.5  ParamDataTypeStr=FOC_Fixed_Config.Types.Coefficient  OutDataTypeStr=FOC_Fixed_Config.Types.Work  RndMeth=Convergent  SaturateOnIntegerOverflow=on
  Elements : Demux  Outputs=2
  Projection : Sum  Inputs=+-  OutDataTypeStr=FOC_Fixed_Config.Types.Work  AccumDataTypeStr=FOC_Fixed_Config.Types.Work  RndMeth=Convergent  SaturateOnIntegerOverflow=on
  Value : Outport
  wires:
  Projection/1 -> Value/1
  Beta05/1 -> Projection/2
  Alpha0866/1 -> Projection/1
  Elements/2 -> Beta05/1
  Elements/1 -> Alpha0866/1
  Vector/1 -> Elements/1

== system gm_PMLSM_FOC_FixedPoint_vnl/FOC_DUT_vnl/SVPWMG/Sector Caculate/B2 ==
  Vector : Inport
  Alpha0866 : Gain  Gain=FOC_Fixed_Config.Coefficients.C0866.quantized  ParamDataTypeStr=FOC_Fixed_Config.Types.Coefficient  OutDataTypeStr=FOC_Fixed_Config.Types.Work  RndMeth=Convergent  SaturateOnIntegerOverflow=on
  Beta05 : Gain  Gain=0.5  ParamDataTypeStr=FOC_Fixed_Config.Types.Coefficient  OutDataTypeStr=FOC_Fixed_Config.Types.Work  RndMeth=Convergent  SaturateOnIntegerOverflow=on
  Elements : Demux  Outputs=2
  Projection : Sum  Inputs=--  OutDataTypeStr=FOC_Fixed_Config.Types.Work  AccumDataTypeStr=FOC_Fixed_Config.Types.Work  RndMeth=Convergent  SaturateOnIntegerOverflow=on
  Value : Outport
  wires:
  Projection/1 -> Value/1
  Beta05/1 -> Projection/2
  Alpha0866/1 -> Projection/1
  Elements/1 -> Alpha0866/1
  Elements/2 -> Beta05/1
  Vector/1 -> Elements/1

== system gm_PMLSM_FOC_FixedPoint_vnl/FOC_DUT_vnl/SVPWMG/Sector Caculate/N ==
  Vector : Inport  OutDataTypeStr=uint8
  Elements : Demux  Outputs=3
  Four : Gain  Gain=4  ParamDataTypeStr=uint8  OutDataTypeStr=uint8  RndMeth=Convergent  SaturateOnIntegerOverflow=on
  SectorNumber : Sum  Inputs=+++  OutDataTypeStr=uint8  AccumDataTypeStr=uint8  RndMeth=Convergent  SaturateOnIntegerOverflow=on
  Two : Gain  Gain=2  ParamDataTypeStr=uint8  OutDataTypeStr=uint8  RndMeth=Convergent  SaturateOnIntegerOverflow=on
  Value : Outport  OutDataTypeStr=uint8
  wires:
  Two/1 -> SectorNumber/2
  Four/1 -> SectorNumber/1
  Elements/2 -> Two/1
  Elements/3 -> Four/1
  Elements/1 -> SectorNumber/3
  SectorNumber/1 -> Value/1
  Vector/1 -> Elements/1

== system gm_PMLSM_FOC_FixedPoint_vnl/FOC_DUT_vnl/SVPWMG/T1T2 Calculate/Fcn ==
  Vector : Inport
  Combination : Sum  Inputs=+--  OutDataTypeStr=FOC_Fixed_Config.Types.Work  AccumDataTypeStr=FOC_Fixed_Config.Types.Work  RndMeth=Convergent  SaturateOnIntegerOverflow=on
  Elements : Demux  Outputs=3
  Value : Outport
  wires:
  Combination/1 -> Value/1
  Elements/3 -> Combination/1
  Elements/2 -> Combination/2
  Elements/1 -> Combination/3
  Vector/1 -> Elements/1

== system gm_PMLSM_FOC_FixedPoint_vnl/FOC_DUT_vnl/SVPWMG/T1T2 Calculate/Fcn1 ==
  Vector : Inport
  Defined_Fallback : Constant  OutDataTypeStr=FOC_Fixed_Config.Types.Work
  Defined_Quotient : Product  Inputs=*/  OutDataTypeStr=FOC_Fixed_Config.Types.Work  RndMeth=Convergent  SaturateOnIntegerOverflow=on
  Denominator_Nonzero : simulink/Logic and Bit Operations/Compare To Zero  relop=~=  OutDataTypeStr=boolean
  Numerator : Product  Inputs=**  OutDataTypeStr=FOC_Fixed_Config.Types.Work  RndMeth=Convergent  SaturateOnIntegerOverflow=on
  Safe_Denominator : Switch  Criteria=u2 ~= 0  OutDataTypeStr=FOC_Fixed_Config.Types.Work  RndMeth=Convergent  InputSameDT=off
  Sum_Times : Sum  OutDataTypeStr=FOC_Fixed_Config.Types.Work  AccumDataTypeStr=FOC_Fixed_Config.Types.Work  RndMeth=Convergent  SaturateOnIntegerOverflow=on
  Times : Demux  Outputs=3
  Value : Outport
  wires:
  Defined_Quotient/1 -> Value/1
  Safe_Denominator/1 -> Defined_Quotient/2
  Defined_Fallback/1 -> Safe_Denominator/3
  Denominator_Nonzero/1 -> Safe_Denominator/2
  Sum_Times/1 -> Denominator_Nonzero/1, Safe_Denominator/1
  Times/3 -> Numerator/2
  Times/2 -> Sum_Times/2
  Numerator/1 -> Defined_Quotient/1
  Vector/1 -> Times/1
  Times/1 -> Numerator/1, Sum_Times/1

== system gm_PMLSM_FOC_FixedPoint_vnl/FOC_DUT_vnl/SVPWMG/T1T2 Calculate/Fcn2 ==
  Vector : Inport
  Defined_Fallback : Constant  OutDataTypeStr=FOC_Fixed_Config.Types.Work
  Defined_Quotient : Product  Inputs=*/  OutDataTypeStr=FOC_Fixed_Config.Types.Work  RndMeth=Convergent  SaturateOnIntegerOverflow=on
  Denominator_Nonzero : simulink/Logic and Bit Operations/Compare To Zero  relop=~=  OutDataTypeStr=boolean
  Numerator : Product  Inputs=**  OutDataTypeStr=FOC_Fixed_Config.Types.Work  RndMeth=Convergent  SaturateOnIntegerOverflow=on
  Safe_Denominator : Switch  Criteria=u2 ~= 0  OutDataTypeStr=FOC_Fixed_Config.Types.Work  RndMeth=Convergent  InputSameDT=off
  Sum_Times : Sum  OutDataTypeStr=FOC_Fixed_Config.Types.Work  AccumDataTypeStr=FOC_Fixed_Config.Types.Work  RndMeth=Convergent  SaturateOnIntegerOverflow=on
  Times : Demux  Outputs=3
  Value : Outport
  wires:
  Defined_Quotient/1 -> Value/1
  Safe_Denominator/1 -> Defined_Quotient/2
  Defined_Fallback/1 -> Safe_Denominator/3
  Denominator_Nonzero/1 -> Safe_Denominator/2
  Sum_Times/1 -> Denominator_Nonzero/1, Safe_Denominator/1
  Numerator/1 -> Defined_Quotient/1
  Times/2 -> Numerator/1, Sum_Times/2
  Times/1 -> Sum_Times/1
  Vector/1 -> Times/1
  Times/3 -> Numerator/2
